simulink model "Full_network_time_optimized"  (R2025b)
settings: Solver=FixedStepAuto  StartTime=0.0  StopTime=30  FixedStep=0.001  RelTol=1e-3
InitFcn:
  | load('FuelPropsData.mat')
libraries: fl_lib x41, nesl_utility x31, SimscapeFluids_lib x13, slpidlib x7, simulink x4
(part 5 of 5)

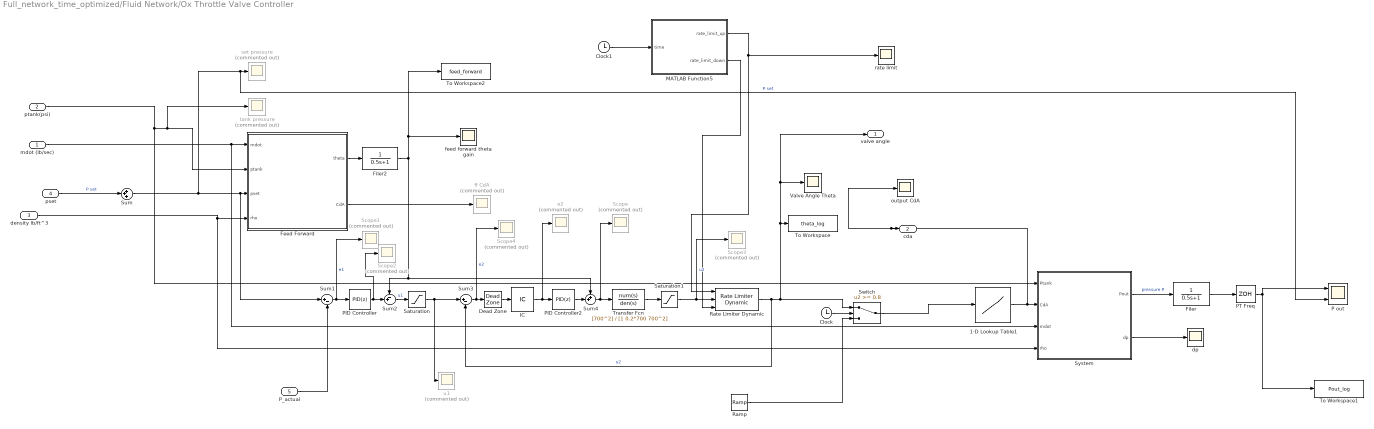
== system Full_network_time_optimized/Fluid Network/Ox Throttle Valve Controller ==
  mdot (lb/sec) : Inport
  ptank(psi) : Inport  Port=2
  density lb/ft^3 : Inport  Port=3
  pset : Inport  Port=4
  P_actual : Inport  Port=5
  1-D Lookup Table1 : Lookup_n-D  NumberOfTableDimensions=1  BreakpointsForDimension1=[27, 36, 45, 54, 63, 72, 81, 90]  Table="[0.01,  0.06, 0.21, 0.46, 0.83, 1.35, 2.04, 2.93] ./ 37.97"  ExtrapMethod=Clip  InternalRulePriority=Speed  RndMeth=Simplest
  Clock : Clock
  Clock1 : Clock
  Dead Zone : DeadZone  LowerValue=-30  UpperValue=30
  Feed Forward : MATLAB Function  TreatAsAtomicUnit=on
  Filer : TransferFcn  Denominator=[0.5 1]
  Filer2 : TransferFcn  Denominator=[0.5 1]
  IC : InitialCondition  Value=0
  MATLAB Function5 : MATLAB Function  TreatAsAtomicUnit=on
  P out : Scope  NumInputPorts=2
      settings: ActiveDisplayYMinimum=-31.526205571372174  ActiveDisplayYMaximum=283.73585014234965  DataLoggingVariableName=ScopeData20
  PID Controller : slpidlib/PID Controller  Controller=PID  Form=Parallel  TimeDomain=Discrete-time  UseExternalTs=off  SampleTime=0.01  IntegratorMethod=Forward Euler  FilterMethod=Forward Euler  ControllerParametersSource=internal  P=6  I=0.5  UseKiTs=off  D=0  UseExternalDerivativeSource=off  N=100  UseFilter=on  TunerSelectOption=Transfer Function Based (PID Tuner App)  InitialConditionSource=internal  InitialConditionForIntegrator=0  InitialConditionForFilter=0  DifferentiatorICPrevScaledInput=0  ExternalReset=none  TrackingMode=off  Kt=1  LimitOutput=off  SatLimitsSource=internal  UpperSaturationLimit=inf  LowerSaturationLimit=-inf  LinearizeAsGain=on  AntiWindupMode=none  Kb=1  LimitIntegrator=off  UpperIntegratorSaturationLimit=inf  LowerIntegratorSaturationLimit=-inf  POutMin=[]  POutMax=[]  IOutMin=[]  IOutMax=[]  DOutMin=[]  DOutMax=[]  NOutMin=[]  NOutMax=[]  SumOutMin=[]  SumOutMax=[]  SaturationOutMin=[]  SaturationOutMax=[]  PParamMin=[]  PParamMax=[]  IParamMin=[]  IParamMax=[]  DParamMin=[]  DParamMax=[]  NParamMin=[]  NParamMax=[]  KbParamMin=[]  KbParamMax=[]  KtParamMin=[]  KtParamMax=[]  KbOutMin=[]  KbOutMax=[]  KtOutMin=[]  KtOutMax=[]  IntegratorOutMin=[]  IntegratorOutMax=[]  FilterOutMin=[]  FilterOutMax=[]  SumI1OutMin=[]  SumI1OutMax=[]  SumI2OutMin=[]  SumI2OutMax=[]  SumI3OutMin=[]  SumI3OutMax=[]  SumI4OutMin=[]  SumI4OutMax=[]  SumDOutMin=[]  SumDOutMax=[]  DifferentiatorOutMin=[]  DifferentiatorOutMax=[]  FilterDiffOutCoefMin=[]  FilterDiffOutCoefMax=[]  ReciprocalOutMin=[]  ReciprocalOutMax=[]  SumDenOutMin=[]  SumDenOutMax=[]  SumNumOutMin=[]  SumNumOutMax=[]  DivideOutMin=[]  DivideOutMax=[]  UdiffTsProdOutMin=[]  UdiffTsProdOutMax=[]  NTsProdOutMin=[]  NTsProdOutMax=[]  UintegralTsProdOutMin=[]  UintegralTsProdOutMax=[]  UngainTsProdOutMin=[]  UngainTsProdOutMax=[]  ClampingZeroOutDataTypeStr=Inherit: Inherit via back propagation  ClampingZeroOutMin=[]  ClampingZeroOutMax=[]  FilterDenConstantOutDataTypeStr=Inherit: Inherit via back propagation  FilterDenConstantOutMin=[]  FilterDenConstantOutMax=[]  PCopyOutDataTypeStr=Inherit: Inherit via back propagation  PCopyOutMin=[]  PCopyOutMax=[]  NCopyOutDataTypeStr=Inherit: Inherit via back propagation  NCopyOutMin=[]  NCopyOutMax=[]  IntegratorContinuousStateAttributes=''  IntegratorStateMustResolveToSignalObject=off  IntegratorRTWStateStorageClass=Auto  FilterContinuousStateAttributes=''  FilterStateMustResolveToSignalObject=off  FilterRTWStateStorageClass=Auto  ParallelPVariant=InternalParameters  IdealPVariant=Disabled  IVariant=InternalParameters  DVariant=InternalParameters  IntegratorVariant=Discrete  SatVariant=Disabled  AWVariant=Passthrough  PCopyVariant=Disabled  TRVariant=Disabled  FdbkBlocksVariant=Forward  IdealPFdbkVariant=Disabled  SatFdbkVariant=Disabled  DerivativeFilterVariant=ForwardEulerFilter  NVariant=InternalParameters  NCopyVariant=Disabled  FilterICVariant=InternalICsFilter  IntegratorICVariant=InternalICs  ExternalResetVariant=Disabled  TRSumVariant=Passthrough  SumFdbkVariant=Disabled  SumVariant=Sum_PID  TsampFilterVariant=InternalTs  TsampNgainVariant=Passthrough  TsampIntegralVariant=Disabled_SignalSpec  ExternalSaturationOutDataTypeStr=Inherit: Same as second input  DerivativeSourceVariant=ErrorSignal  PreIntVariant=InternalPreInt
  PID Controller2 : slpidlib/PID Controller  Controller=PID  Form=Parallel  TimeDomain=Discrete-time  UseExternalTs=off  SampleTime=0.001  IntegratorMethod=Forward Euler  FilterMethod=Forward Euler  ControllerParametersSource=internal  P=0.1  I=0.6  UseKiTs=off  D=0  UseExternalDerivativeSource=off  N=100  UseFilter=on  TunerSelectOption=Transfer Function Based (PID Tuner App)  InitialConditionSource=internal  InitialConditionForIntegrator=0  InitialConditionForFilter=0  DifferentiatorICPrevScaledInput=0  ExternalReset=none  TrackingMode=off  Kt=1  LimitOutput=off  SatLimitsSource=internal  UpperSaturationLimit=inf  LowerSaturationLimit=-inf  LinearizeAsGain=on  AntiWindupMode=none  Kb=1  LimitIntegrator=off  UpperIntegratorSaturationLimit=inf  LowerIntegratorSaturationLimit=-inf  POutMin=[]  POutMax=[]  IOutMin=[]  IOutMax=[]  DOutMin=[]  DOutMax=[]  NOutMin=[]  NOutMax=[]  SumOutMin=[]  SumOutMax=[]  SaturationOutMin=[]  SaturationOutMax=[]  PParamMin=[]  PParamMax=[]  IParamMin=[]  IParamMax=[]  DParamMin=[]  DParamMax=[]  NParamMin=[]  NParamMax=[]  KbParamMin=[]  KbParamMax=[]  KtParamMin=[]  KtParamMax=[]  KbOutMin=[]  KbOutMax=[]  KtOutMin=[]  KtOutMax=[]  IntegratorOutMin=[]  IntegratorOutMax=[]  FilterOutMin=[]  FilterOutMax=[]  SumI1OutMin=[]  SumI1OutMax=[]  SumI2OutMin=[]  SumI2OutMax=[]  SumI3OutMin=[]  SumI3OutMax=[]  SumI4OutMin=[]  SumI4OutMax=[]  SumDOutMin=[]  SumDOutMax=[]  DifferentiatorOutMin=[]  DifferentiatorOutMax=[]  FilterDiffOutCoefMin=[]  FilterDiffOutCoefMax=[]  ReciprocalOutMin=[]  ReciprocalOutMax=[]  SumDenOutMin=[]  SumDenOutMax=[]  SumNumOutMin=[]  SumNumOutMax=[]  DivideOutMin=[]  DivideOutMax=[]  UdiffTsProdOutMin=[]  UdiffTsProdOutMax=[]  NTsProdOutMin=[]  NTsProdOutMax=[]  UintegralTsProdOutMin=[]  UintegralTsProdOutMax=[]  UngainTsProdOutMin=[]  UngainTsProdOutMax=[]  ClampingZeroOutDataTypeStr=Inherit: Inherit via back propagation  ClampingZeroOutMin=[]  ClampingZeroOutMax=[]  FilterDenConstantOutDataTypeStr=Inherit: Inherit via back propagation  FilterDenConstantOutMin=[]  FilterDenConstantOutMax=[]  PCopyOutDataTypeStr=Inherit: Inherit via back propagation  PCopyOutMin=[]  PCopyOutMax=[]  NCopyOutDataTypeStr=Inherit: Inherit via back propagation  NCopyOutMin=[]  NCopyOutMax=[]  IntegratorContinuousStateAttributes=''  IntegratorStateMustResolveToSignalObject=off  IntegratorRTWStateStorageClass=Auto  FilterContinuousStateAttributes=''  FilterStateMustResolveToSignalObject=off  FilterRTWStateStorageClass=Auto  ParallelPVariant=InternalParameters  IdealPVariant=Disabled  IVariant=InternalParameters  DVariant=InternalParameters  IntegratorVariant=Discrete  SatVariant=Disabled  AWVariant=Passthrough  PCopyVariant=Disabled  TRVariant=Disabled  FdbkBlocksVariant=Forward  IdealPFdbkVariant=Disabled  SatFdbkVariant=Disabled  DerivativeFilterVariant=ForwardEulerFilter  NVariant=InternalParameters  NCopyVariant=Disabled  FilterICVariant=InternalICsFilter  IntegratorICVariant=InternalICs  ExternalResetVariant=Disabled  TRSumVariant=Passthrough  SumFdbkVariant=Disabled  SumVariant=Sum_PID  TsampFilterVariant=InternalTs  TsampNgainVariant=Passthrough  TsampIntegralVariant=Disabled_SignalSpec  ExternalSaturationOutDataTypeStr=Inherit: Same as second input  DerivativeSourceVariant=ErrorSignal  PreIntVariant=InternalPreInt
  PT Freq : ZeroOrderHold  SampleTime=1/200
  Ramp : simulink/Sources/Ramp  slope=48  start=0  InitialOutput=0
  Rate Limiter Dynamic : simulink/Discontinuities/Rate Limiter Dynamic
  Saturation : Saturate  UpperLimit=90  LowerLimit=0
  Saturation1 : Saturate  UpperLimit=90  LowerLimit=0
  Scope{,1..4} (5 alike) : Scope  Commented=on
      Scope settings: ActiveDisplayYMinimum=-275.11641924282065  ActiveDisplayYMaximum=563.35245614782866  DataLoggingVariableName=ScopeData23
      Scope1 settings: ActiveDisplayYMinimum=-63.640747784829  ActiveDisplayYMaximum=395.9600830872032  DataLoggingVariableName=ScopeData24
      Scope2 settings: ActiveDisplayYMinimum=-1  ActiveDisplayYMaximum=1  DataLoggingVariableName=ScopeData25
      Scope3 settings: ActiveDisplayYMinimum=-1  ActiveDisplayYMaximum=1  DataLoggingVariableName=ScopeData26
      Scope4 settings: ActiveDisplayYMinimum=-1  ActiveDisplayYMaximum=1  DataLoggingVariableName=ScopeData27
  Sum : Sum  Inputs=+++
  Sum1 : Sum  Inputs=|+-
  Sum2 : Sum  Inputs=-+|
  Sum3 : Sum  Inputs=|+-
  Sum4 : Sum  Inputs=++|
  Switch : Switch  Threshold=0.8  SaturateOnIntegerOverflow=off  InputSameDT=off
  System : MATLAB Function  TreatAsAtomicUnit=on
  To Workspace : ToWorkspace  VariableName=theta_log  SampleTime=-1
  To Workspace1 : ToWorkspace  VariableName=Pout_log  SaveFormat=Structure With Time  SampleTime=-1
  To Workspace2 : ToWorkspace  VariableName=feed_forward  SampleTime=-1
  Transfer Fcn : TransferFcn  Numerator=[700^2]  Denominator=[1 0.2*700 700^2]
  Valve Angle Theta : Scope
      settings: ActiveDisplayYMinimum=-6.3882474794481388  ActiveDisplayYMaximum=57.494227315033264
  dp : Scope
      settings: ActiveDisplayYMinimum=-1  ActiveDisplayYMaximum=1  DataLoggingVariableName=ScopeData28
  e2 : Scope  Commented=on
      settings: ActiveDisplayYMinimum=-94.713391249832966  ActiveDisplayYMaximum=253.61308310962266  DataLoggingVariableName=ScopeData29
  feed forward theta gain : Scope
      settings: ActiveDisplayYMinimum=36.144112332478429  ActiveDisplayYMaximum=40.8018145520034  DataLoggingVariableName=ScopeData2
  ff CdA : Scope  Commented=on
      settings: ActiveDisplayYMinimum=0.00619  ActiveDisplayYMaximum=0.00757  DataLoggingVariableName=ScopeData30
  output CdA : Scope
      settings: ActiveDisplayYMinimum=-0.00091146165836572817  ActiveDisplayYMaximum=0.010836813076463534  DataLoggingVariableName=ScopeData3
  rate limit : Scope
      settings: ActiveDisplayYMinimum=-123.74999999999997  ActiveDisplayYMaximum=1513.75  DataLoggingVariableName=ScopeData31
  set pressure : Scope  Commented=on
      settings: ActiveDisplayYMinimum=-1  ActiveDisplayYMaximum=1  DataLoggingVariableName=ScopeData32
  tank pressure : Scope  Commented=on
      settings: ActiveDisplayYMinimum=243.75  ActiveDisplayYMaximum=306.25  DataLoggingVariableName=ScopeData33
  u1 : Scope  Commented=on
      settings: ActiveDisplayYMinimum=-1  ActiveDisplayYMaximum=1  DataLoggingVariableName=ScopeData34
  valve angle : Outport
  cda : Outport  Port=2
  wires:
  Sum3/1 -> Dead Zone/1, Scope4/1  "e2"
  density lb/ft^3/1 -> System/4(rho), Feed Forward/4(rho)
  Filer/1 -> PT Freq/1
  Sum/1 -> P out/2, set pressure/1, Sum1/1, Feed Forward/3(pset)  "P set"
  ptank(psi)/1 -> System/1(Ptank), Feed Forward/2(ptank), tank pressure/1
  PID Controller/1 -> Scope2/1, Sum2/2
  PT Freq/1 -> P out/1, To Workspace1/1
  Transfer Fcn/1 -> Saturation1/1
  IC/1 -> PID Controller2/1, e2/1
  Feed Forward/1(theta) -> Filer2/1
  MATLAB Function5/2(rate_limit_down) -> Rate Limiter Dynamic/3
  Dead Zone/1 -> IC/1
  Rate Limiter Dynamic/1 -> Switch/1, valve angle/1, Valve Angle Theta/1, To Workspace/1, Sum3/2  "u2"
  pset/1 -> Sum/2  "P set"
  Sum4/1 -> Scope/1, Transfer Fcn/1
  Saturation1/1 -> Scope3/1, Rate Limiter Dynamic/2  "u2"
  mdot (lb/sec)/1 -> System/3(mdot), Feed Forward/1(mdot)
  MATLAB Function5/1(rate_limit_up) -> Rate Limiter Dynamic/1, rate limit/1
  Clock1/1 -> MATLAB Function5/1(time)
  1-D Lookup Table1/1 -> System/2(CdA), output CdA/1, cda/1
  PID Controller2/1 -> Sum4/2
  Sum1/1 -> Scope1/1, PID Controller/1  "e1"
  Sum2/1 -> Saturation/1  "u1"
  Feed Forward/2(CdA) -> ff CdA/1
  System/2(dp) -> dp/1
  Saturation/1 -> u1/1, Sum3/1
  System/1(Pout) -> Filer/1  "pressure P"
  Filer2/1 -> Sum4/1, Sum2/1, feed forward theta gain/1, To Workspace2/1
  P_actual/1 -> Sum1/2
  Clock/1 -> Switch/2
  Ramp/1 -> Switch/3
  Switch/1 -> 1-D Lookup Table1/1

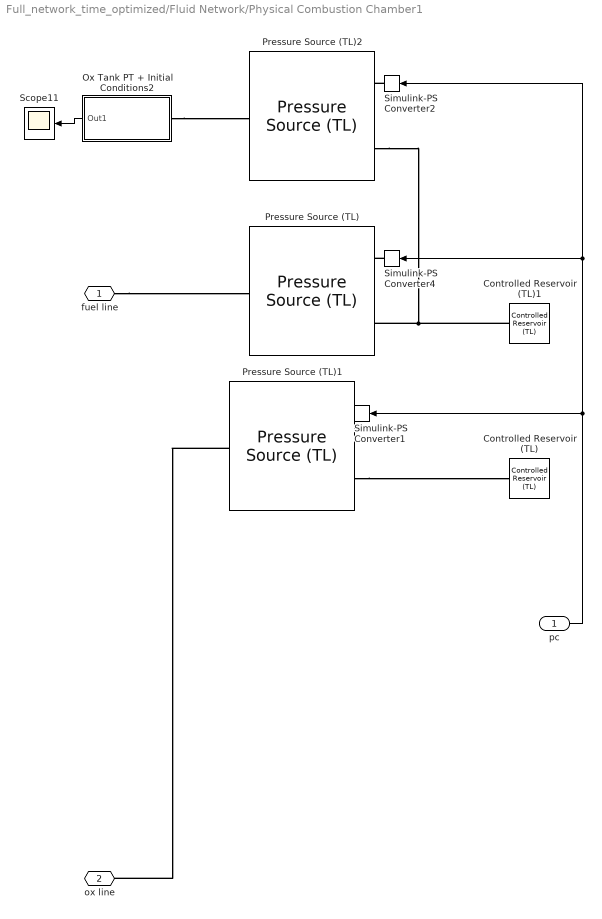
== system Full_network_time_optimized/Fluid Network/Physical Combustion Chamber1 ==
  pc : Inport
  Controlled Reservoir (TL) : fl_lib/Thermal Liquid/Elements/Controlled Reservoir (TL)  pressure_spec=foundation.enum.pressure_spec.atmospheric  reservoir_pressure=0.101325 MPa  area=0.01 m^2
      settings: InternalSimscapePortConfiguration="{\"Bottom\":[],\"Left\":[{\"id\":\"A\",\"label\":\"A\",\"type\":\"foundation.thermal_liquid.thermal_liquid\"}],\"Right\":[{\"id\":\"T_in\",\"label\":\"T\",\"type\":\"input\"}],\"Top\":[]}"
  Controlled Reservoir (TL)1 : fl_lib/Thermal Liquid/Elements/Controlled Reservoir (TL)  pressure_spec=foundation.enum.pressure_spec.atmospheric  reservoir_pressure=0.101325 MPa  area=0.01 m^2
      settings: InternalSimscapePortConfiguration="{\"Bottom\":[],\"Left\":[{\"id\":\"A\",\"label\":\"A\",\"type\":\"foundation.thermal_liquid.thermal_liquid\"}],\"Right\":[{\"id\":\"T_in\",\"label\":\"T\",\"type\":\"input\"}],\"Top\":[]}"
  Ox Tank PT + Initial Conditions2 : Subsystem
  Pressure Source (TL) : fl_lib/Thermal Liquid/Sources/Pressure Source (TL)  source_type=foundation.enum.constant_controlled.controlled  pressure_differential=0 MPa  power_spec=foundation.enum.power_spec.isentropic  area=0.01 m^2
      settings: InternalSimscapePortConfiguration="{\"Bottom\":[],\"Left\":[{\"id\":\"A\",\"label\":\"A\",\"type\":\"foundation.thermal_liquid.thermal_liquid\"},{\"id\":\"P\",\"label\":\"P\",\"type\":\"input\"}],\"Right\":[{\"id\":\"B\",\"label\":\"B\",\"type\":\"foundation.thermal_liquid.thermal_liquid\"}],\"Top\":[]}"
  Pressure Source (TL)1 : fl_lib/Thermal Liquid/Sources/Pressure Source (TL)  source_type=foundation.enum.constant_controlled.controlled  pressure_differential=0 MPa  power_spec=foundation.enum.power_spec.isentropic  area=0.01 m^2
      settings: InternalSimscapePortConfiguration="{\"Bottom\":[],\"Left\":[{\"id\":\"A\",\"label\":\"A\",\"type\":\"foundation.thermal_liquid.thermal_liquid\"},{\"id\":\"P\",\"label\":\"P\",\"type\":\"input\"}],\"Right\":[{\"id\":\"B\",\"label\":\"B\",\"type\":\"foundation.thermal_liquid.thermal_liquid\"}],\"Top\":[]}"
  Pressure Source (TL)2 : fl_lib/Thermal Liquid/Sources/Pressure Source (TL)  source_type=foundation.enum.constant_controlled.controlled  pressure_differential=0 MPa  power_spec=foundation.enum.power_spec.isentropic  area=0.01 m^2
      settings: InternalSimscapePortConfiguration="{\"Bottom\":[],\"Left\":[{\"id\":\"A\",\"label\":\"A\",\"type\":\"foundation.thermal_liquid.thermal_liquid\"},{\"id\":\"P\",\"label\":\"P\",\"type\":\"input\"}],\"Right\":[{\"id\":\"B\",\"label\":\"B\",\"type\":\"foundation.thermal_liquid.thermal_liquid\"}],\"Top\":[]}"
  Scope11 : Scope
      settings: ActiveDisplayYMinimum=-62.499971643181354  ActiveDisplayYMaximum=562.49999684924239  DataLoggingVariableName=ScopeData48
  Simulink-PS Converter1 : nesl_utility/Simulink-PS Converter  PhysicalDomain=network_engine_domain  SubClassName=ps_input  LeftPortType=input  RightPortType=output  PseudoPeriodic=off  Frequencies=[]  NoiseDistribution=none  NoiseParameters=[]  Unit=1  AffineConversion=off  FilteringAndDerivatives=filter  SimscapeFilterOrder=1  InputFilterTimeConstant=0.001  UdotUserProvided=0
  Simulink-PS Converter2 : nesl_utility/Simulink-PS Converter  PhysicalDomain=network_engine_domain  SubClassName=ps_input  LeftPortType=input  RightPortType=output  PseudoPeriodic=off  Frequencies=[]  NoiseDistribution=none  NoiseParameters=[]  Unit=1  AffineConversion=off  FilteringAndDerivatives=filter  SimscapeFilterOrder=1  InputFilterTimeConstant=0.001  UdotUserProvided=0
  Simulink-PS Converter4 : nesl_utility/Simulink-PS Converter  PhysicalDomain=network_engine_domain  SubClassName=ps_input  LeftPortType=input  RightPortType=output  PseudoPeriodic=off  Frequencies=[]  NoiseDistribution=none  NoiseParameters=[]  Unit=1  AffineConversion=off  FilteringAndDerivatives=filter  SimscapeFilterOrder=1  InputFilterTimeConstant=0.001  UdotUserProvided=0
  fuel line : PMIOPort  Side=Right
  ox line : PMIOPort  Port=2  Side=Right
  wires:
  pc/1 -> Simulink-PS Converter1/1, Simulink-PS Converter2/1, Simulink-PS Converter4/1
  Ox Tank PT + Initial Conditions2/1(Out1) -> Scope11/1
  connections:
  Simulink-PS Converter4/RConn1 -- Pressure Source (TL)/LConn2
  Simulink-PS Converter1/RConn1 -- Pressure Source (TL)1/LConn2
  Controlled Reservoir (TL)1/LConn1 -- Pressure Source (TL)2/LConn1 -- Pressure Source (TL)/LConn1
  fuel line/RConn1 -- Pressure Source (TL)/RConn1
  Pressure Source (TL)1/RConn1 -- ox line/RConn1
  Pressure Source (TL)1/LConn1 -- Controlled Reservoir (TL)/LConn1
  Simulink-PS Converter2/RConn1 -- Pressure Source (TL)2/LConn2
  Ox Tank PT + Initial Conditions2/LConn1 -- Pressure Source (TL)2/RConn1

== system Full_network_time_optimized/Fluid Network/fuel mdot feedback//corrections ==
  actual mdot : Inport
  commanded mdot : Inport  Port=2
  MR correction : Inport  Port=3
  PID Controller1 : slpidlib/PID Controller  Controller=PID  Form=Parallel  TimeDomain=Continuous-time  UseExternalTs=off  SampleTime=-1  IntegratorMethod=Forward Euler  FilterMethod=Forward Euler  ControllerParametersSource=internal  P=1  I=0  UseKiTs=off  D=0  UseExternalDerivativeSource=off  N=20  UseFilter=on  TunerSelectOption=Transfer Function Based (PID Tuner App)  InitialConditionSource=internal  InitialConditionForIntegrator=0  InitialConditionForFilter=0  DifferentiatorICPrevScaledInput=0  ExternalReset=none  TrackingMode=off  Kt=1  LimitOutput=off  SatLimitsSource=internal  UpperSaturationLimit=inf  LowerSaturationLimit=-inf  LinearizeAsGain=on  AntiWindupMode=none  Kb=1  LimitIntegrator=off  UpperIntegratorSaturationLimit=inf  LowerIntegratorSaturationLimit=-inf  POutMin=[]  POutMax=[]  IOutMin=[]  IOutMax=[]  DOutMin=[]  DOutMax=[]  NOutMin=[]  NOutMax=[]  SumOutMin=[]  SumOutMax=[]  SaturationOutMin=[]  SaturationOutMax=[]  PParamMin=[]  PParamMax=[]  IParamMin=[]  IParamMax=[]  DParamMin=[]  DParamMax=[]  NParamMin=[]  NParamMax=[]  KbParamMin=[]  KbParamMax=[]  KtParamMin=[]  KtParamMax=[]  KbOutMin=[]  KbOutMax=[]  KtOutMin=[]  KtOutMax=[]  IntegratorOutMin=[]  IntegratorOutMax=[]  FilterOutMin=[]  FilterOutMax=[]  SumI1OutMin=[]  SumI1OutMax=[]  SumI2OutMin=[]  SumI2OutMax=[]  SumI3OutMin=[]  SumI3OutMax=[]  SumI4OutMin=[]  SumI4OutMax=[]  SumDOutMin=[]  SumDOutMax=[]  DifferentiatorOutMin=[]  DifferentiatorOutMax=[]  FilterDiffOutCoefMin=[]  FilterDiffOutCoefMax=[]  ReciprocalOutMin=[]  ReciprocalOutMax=[]  SumDenOutMin=[]  SumDenOutMax=[]  SumNumOutMin=[]  SumNumOutMax=[]  DivideOutMin=[]  DivideOutMax=[]  UdiffTsProdOutMin=[]  UdiffTsProdOutMax=[]  NTsProdOutMin=[]  NTsProdOutMax=[]  UintegralTsProdOutMin=[]  UintegralTsProdOutMax=[]  UngainTsProdOutMin=[]  UngainTsProdOutMax=[]  ClampingZeroOutDataTypeStr=Inherit: Inherit via back propagation  ClampingZeroOutMin=[]  ClampingZeroOutMax=[]  FilterDenConstantOutDataTypeStr=Inherit: Inherit via back propagation  FilterDenConstantOutMin=[]  FilterDenConstantOutMax=[]  PCopyOutDataTypeStr=Inherit: Inherit via back propagation  PCopyOutMin=[]  PCopyOutMax=[]  NCopyOutDataTypeStr=Inherit: Inherit via back propagation  NCopyOutMin=[]  NCopyOutMax=[]  IntegratorContinuousStateAttributes=''  IntegratorStateMustResolveToSignalObject=off  IntegratorRTWStateStorageClass=Auto  FilterContinuousStateAttributes=''  FilterStateMustResolveToSignalObject=off  FilterRTWStateStorageClass=Auto  ParallelPVariant=InternalParameters  IdealPVariant=Disabled  IVariant=InternalParameters  DVariant=InternalParameters  IntegratorVariant=Continuous  SatVariant=Disabled  AWVariant=Passthrough  PCopyVariant=Disabled  TRVariant=Disabled  FdbkBlocksVariant=Forward  IdealPFdbkVariant=Disabled  SatFdbkVariant=Disabled  DerivativeFilterVariant=ContFilter  NVariant=InternalParameters  NCopyVariant=Disabled  FilterICVariant=InternalICsFilter  IntegratorICVariant=InternalICs  ExternalResetVariant=Disabled  TRSumVariant=Passthrough  SumFdbkVariant=Disabled  SumVariant=Sum_PID  TsampFilterVariant=InternalTs  TsampNgainVariant=Passthrough  TsampIntegralVariant=Disabled_SignalSpec  ExternalSaturationOutDataTypeStr=Inherit: Same as second input  DerivativeSourceVariant=ErrorSignal  PreIntVariant=InternalPreInt
  Sum2 : Sum  Inputs=|+-
  Sum3 : Sum  Inputs=|+-
  Sum4 : Sum  Inputs=|++
  kg/s to lb/s1 : Gain  Gain=2.20462
  fuel mdot : Outport
  wires:
  PID Controller1/1 -> Sum4/1
  Sum3/1 -> PID Controller1/1
  Sum4/1 -> kg/s to lb/s1/1
  commanded mdot/1 -> Sum2/1
  Sum2/1 -> Sum3/1
  MR correction/1 -> Sum3/2
  kg/s to lb/s1/1 -> fuel mdot/1

== system Full_network_time_optimized/Fluid Network/ox mdot feedback//corrections ==
  commanded mdot : Inport
  actual mdot : Inport  Port=2
  PID Controller2 : slpidlib/PID Controller  Commented=through  Controller=PID  Form=Parallel  TimeDomain=Continuous-time  UseExternalTs=off  SampleTime=-1  IntegratorMethod=Forward Euler  FilterMethod=Forward Euler  ControllerParametersSource=internal  P=1  I=0  UseKiTs=off  D=0  UseExternalDerivativeSource=off  N=20  UseFilter=on  TunerSelectOption=Transfer Function Based (PID Tuner App)  InitialConditionSource=internal  InitialConditionForIntegrator=0  InitialConditionForFilter=0  DifferentiatorICPrevScaledInput=0  ExternalReset=none  TrackingMode=off  Kt=1  LimitOutput=off  SatLimitsSource=internal  UpperSaturationLimit=inf  LowerSaturationLimit=-inf  LinearizeAsGain=on  AntiWindupMode=none  Kb=1  LimitIntegrator=off  UpperIntegratorSaturationLimit=inf  LowerIntegratorSaturationLimit=-inf  POutMin=[]  POutMax=[]  IOutMin=[]  IOutMax=[]  DOutMin=[]  DOutMax=[]  NOutMin=[]  NOutMax=[]  SumOutMin=[]  SumOutMax=[]  SaturationOutMin=[]  SaturationOutMax=[]  PParamMin=[]  PParamMax=[]  IParamMin=[]  IParamMax=[]  DParamMin=[]  DParamMax=[]  NParamMin=[]  NParamMax=[]  KbParamMin=[]  KbParamMax=[]  KtParamMin=[]  KtParamMax=[]  KbOutMin=[]  KbOutMax=[]  KtOutMin=[]  KtOutMax=[]  IntegratorOutMin=[]  IntegratorOutMax=[]  FilterOutMin=[]  FilterOutMax=[]  SumI1OutMin=[]  SumI1OutMax=[]  SumI2OutMin=[]  SumI2OutMax=[]  SumI3OutMin=[]  SumI3OutMax=[]  SumI4OutMin=[]  SumI4OutMax=[]  SumDOutMin=[]  SumDOutMax=[]  DifferentiatorOutMin=[]  DifferentiatorOutMax=[]  FilterDiffOutCoefMin=[]  FilterDiffOutCoefMax=[]  ReciprocalOutMin=[]  ReciprocalOutMax=[]  SumDenOutMin=[]  SumDenOutMax=[]  SumNumOutMin=[]  SumNumOutMax=[]  DivideOutMin=[]  DivideOutMax=[]  UdiffTsProdOutMin=[]  UdiffTsProdOutMax=[]  NTsProdOutMin=[]  NTsProdOutMax=[]  UintegralTsProdOutMin=[]  UintegralTsProdOutMax=[]  UngainTsProdOutMin=[]  UngainTsProdOutMax=[]  ClampingZeroOutDataTypeStr=Inherit: Inherit via back propagation  ClampingZeroOutMin=[]  ClampingZeroOutMax=[]  FilterDenConstantOutDataTypeStr=Inherit: Inherit via back propagation  FilterDenConstantOutMin=[]  FilterDenConstantOutMax=[]  PCopyOutDataTypeStr=Inherit: Inherit via back propagation  PCopyOutMin=[]  PCopyOutMax=[]  NCopyOutDataTypeStr=Inherit: Inherit via back propagation  NCopyOutMin=[]  NCopyOutMax=[]  IntegratorContinuousStateAttributes=''  IntegratorStateMustResolveToSignalObject=off  IntegratorRTWStateStorageClass=Auto  FilterContinuousStateAttributes=''  FilterStateMustResolveToSignalObject=off  FilterRTWStateStorageClass=Auto  ParallelPVariant=InternalParameters  IdealPVariant=Disabled  IVariant=InternalParameters  DVariant=InternalParameters  IntegratorVariant=Continuous  SatVariant=Disabled  AWVariant=Passthrough  PCopyVariant=Disabled  TRVariant=Disabled  FdbkBlocksVariant=Forward  IdealPFdbkVariant=Disabled  SatFdbkVariant=Disabled  DerivativeFilterVariant=ContFilter  NVariant=InternalParameters  NCopyVariant=Disabled  FilterICVariant=InternalICsFilter  IntegratorICVariant=InternalICs  ExternalResetVariant=Disabled  TRSumVariant=Passthrough  SumFdbkVariant=Disabled  SumVariant=Sum_PID  TsampFilterVariant=InternalTs  TsampNgainVariant=Passthrough  TsampIntegralVariant=Disabled_SignalSpec  ExternalSaturationOutDataTypeStr=Inherit: Same as second input  DerivativeSourceVariant=ErrorSignal  PreIntVariant=InternalPreInt
  Sum1 : Sum  Inputs=|+-
  Sum5 : Sum  Inputs=|++
  kg/s to lb/s : Gain  Gain=2.20462
  ox mdot : Outport
  wires:
  Sum1/1 -> PID Controller2/1
  commanded mdot/1 -> Sum1/1
  PID Controller2/1 -> Sum5/1
  Sum5/1 -> kg/s to lb/s/1
  kg/s to lb/s/1 -> ox mdot/1

== system Full_network_time_optimized/Fluid Network/COPV/COPV Leakage ==
  Leak Rate : fl_lib/Gas/Elements/Flow Resistance (G)  delta_p_nominal=0.001 MPa  mdot_nominal=0.0000000001 kg/s  rho_nominal=0 kg/m^3  area=0.01 m^2  laminar_fraction=1e-3
      settings: InternalSimscapePortConfiguration="{\"Bottom\":[],\"Left\":[{\"id\":\"A\",\"label\":\"A\",\"type\":\"foundation.gas.gas\"}],\"Right\":[{\"id\":\"B\",\"label\":\"B\",\"type\":\"foundation.gas.gas\"}],\"Top\":[]}"
  Mass & Energy Flow Rate Sensor (G)2 : fl_lib/Gas/Sensors/Flow Rate Sensor (G)  mass_flow_measure=true  volumetric_flow_measure=false  volumetric_flow_conditions=foundation.enum.volumetric_flow_conditions.actual  p_std=0.101325 MPa  T_std=20 degC  energy_flow_measure=true
      settings: InternalSimscapePortConfiguration="{\"Bottom\":[{\"id\":\"PHI\",\"label\":\"φ\",\"type\":\"output\"}],\"Left\":[{\"id\":\"A\",\"label\":\"A\",\"type\":\"foundation.gas.gas\"}],\"Right\":[{\"id\":\"B\",\"label\":\"B\",\"type\":\"foundation.gas.gas\"},{\"id\":\"M\",\"label\":\"M\",\"type\":\"output\"}],\"Top\":[]}"
  PS-Simulink Converter7 : nesl_utility/PS-Simulink Converter  PhysicalDomain=network_engine_domain  SubClassName=ps_output  LeftPortType=input  RightPortType=output  PseudoPeriodic=off  Frequencies=[]  VectorFormat=inherit  Unit=inherit  AffineConversion=off
  Pressurant Mass Leak Rate : Scope  Commented=on
      settings: ActiveDisplayYMinimum=-1  ActiveDisplayYMaximum=1
  Reservoir (G) : fl_lib/Gas/Elements/Reservoir (G)  pressure_spec=foundation.enum.pressure_spec.atmospheric  reservoir_pressure=0.101325 MPa  reservoir_temperature=293.15 K  area_A=0.01 m^2
  Conn1 : PMIOPort  Side=Right
  wires:
  PS-Simulink Converter7/1 -> Pressurant Mass Leak Rate/1
  connections:
  Conn1/RConn1 -- Leak Rate/RConn1
  Leak Rate/LConn1 -- Mass & Energy Flow Rate Sensor (G)2/LConn1
  Mass & Energy Flow Rate Sensor (G)2/RConn1 -- Reservoir (G)/LConn1
  Mass & Energy Flow Rate Sensor (G)2/RConn2 -- PS-Simulink Converter7/LConn1

== system Full_network_time_optimized/Fluid Network/Physical Combustion Chamber1/Ox Tank PT + Initial Conditions2 ==
  Initial OT Pressure : InitialCondition  Value=500
  PS-Simulink Converter3 : nesl_utility/PS-Simulink Converter  PhysicalDomain=network_engine_domain  SubClassName=ps_output  LeftPortType=input  RightPortType=output  PseudoPeriodic=off  Frequencies=[]  VectorFormat=inherit  Unit=inherit  AffineConversion=off
  Pa to psi : Gain  Gain=0.000145038
  Pressure & Temperature Sensor (TL) : fl_lib/Thermal Liquid/Sensors/Pressure & Temperature Sensor (TL)  reference=foundation.enum.MeasurementReference.absolute  pressure=true  pressure_spec=foundation.enum.PressureMeasementSpec.Gauge  temperature=false
      settings: InternalSimscapePortConfiguration="{\"Bottom\":[],\"Left\":[{\"id\":\"A\",\"label\":\"A\",\"type\":\"foundation.thermal_liquid.thermal_liquid\"}],\"Right\":[{\"id\":\"Pg\",\"label\":\"Pg\",\"type\":\"output\"}],\"Top\":[]}"
  fuel line : PMIOPort  Side=Left
  Out1 : Outport
  wires:
  Initial OT Pressure/1 -> Out1/1
  Pa to psi/1 -> Initial OT Pressure/1
  PS-Simulink Converter3/1 -> Pa to psi/1
  connections:
  PS-Simulink Converter3/LConn1 -- Pressure & Temperature Sensor (TL)/RConn1
  Pressure & Temperature Sensor (TL)/LConn1 -- fuel line/RConn1

== matlab function Full_network_time_optimized/Fluid Network/Fuel Throttle Valve Controller/MATLAB Function5 ==
  data: time input; rate_limit_up output; rate_limit_down output
function [rate_limit_up, rate_limit_down] = fcn(time)
if time < 0.5
    rate_limit_up = 1350;
else
    rate_limit_up = 40;
end
rate_limit_down = -rate_limit_up;

== matlab function Full_network_time_optimized/Fluid Network/Fuel Throttle Valve Controller/System ==
  data: Ptank input; CdA input; mdot input; Pout output; rho input; dp output
function [Pout,dp] = theta_to_pressure(Ptank,CdA,mdot, rho)

% CdA = mdot/(sqrt((2*(ptank-pout)*rho)

%CdA = max(CdA, 1e-7);
dp = (mdot/CdA)^2*1/(2*rho);

% (mdot/CdA)^2*rho/2 is solving for the pout from the dp in CdA eqn
Pout = Ptank - dp;
Pout = max(Pout, 0);

== matlab function Full_network_time_optimized/Fluid Network/Injector1/Fuel Injector Calculations ==
  data: P_down input; rho input; mdot input; CdA input; stiffness output; P_up output; dP_inj output
function [stiffness, P_up, dP_inj] = injectorModel(P_down, rho, mdot, CdA)
%#codegen
% Injector model using known downstream pressure, density, mdot, and CdA
%
% Inputs:
%   P_down - Downstream / chamber pressure [Pa]
%   rho    - Fluid density [kg/m^3]
%   mdot   - Mass flow rate through injector [kg/s]
%   CdA    - Effective injector area, Cd*A [m^2]
%
% Outputs:
%   stiffness - Injector stiffness, S = dP_inj / P_down [-]
%   P_up      - Required upstream / manifold pressure [Pa]
%   dP_inj    - Pressure drop across injector [Pa]
%
% Equations:
%   mdot   = CdA * sqrt(2 * rho * dP_inj)
%   => dP_inj = (mdot / CdA)^2 / (2*rho)
%
%   P_up = P_down + dP_inj
%   stiffness = dP_inj / P_down

    % Compute pressure drop from orifice equation
    dP_inj = (mdot / CdA)^2 / (2 * rho);

    % Upstream pressure
    P_up = P_down + dP_inj;

    % Stiffness
    stiffness = dP_inj / P_down;

end

== matlab function Full_network_time_optimized/Fluid Network/Thrust Commanded to mdot + bunch of other bs ==
  data: mdot_fuel output; rho_fuel_eng output; pc output; F_cmd input; rho_ox input; rho_fuel input; rho_ox_eng output; mdot_ox output; Cf input; MR input; cstar_ideal input; cstar_eff input
function [mdot_fuel, rho_fuel_eng, pc, rho_ox_eng, mdot_ox] = thrust_to_mdot( ...
   F_cmd, rho_ox, rho_fuel, Cf, MR, cstar_ideal, cstar_eff)
%#codegen
% Convert commanded thrust into mdots and convert densities to English units
%
% Outputs:
%   mdot_ox        - oxidizer mass flow rate [kg/s]
%   mdot_fuel      - fuel mass flow rate [kg/s]
%   rho_ox_eng     - oxidizer density [lb/ft^3]
%   rho_fuel_eng   - fuel density [lb/ft^3]
%   mdot_ox_lb     - oxidizer mass flow rate [lb/s]
%   mdot_fuel_lb   - fuel mass flow rate [lb/s]

    cstar = cstar_ideal * cstar_eff;
    At = 0.0008271;      % throat area [m^2]

    %% ---- DEFAULT OUTPUTS ----
    mdot_ox = 0;
    mdot_fuel = 0;
    rho_ox_eng = 0;
    rho_fuel_eng = 0;
    mdot_ox_lb = 0;
    mdot_fuel_lb = 0;

    %% ---- UNIT CONVERSION ----
    kgm3_to_lbft3 = 0.062428;
    kg_to_lb = 2.20462;

    rho_ox_eng = rho_ox * kgm3_to_lbft3;
    rho_fuel_eng = rho_fuel * kgm3_to_lbft3;

    %% ---- EFFECTIVE EXHAUST VELOCITY ----
    ve = Cf * cstar;


    %% ---- TOTAL MASS FLOW ----
    mdot_total = F_cmd / ve;

    pc = mdot_total * cstar / At;

    pc = pc * 0.000145038;

    %% ---- SPLIT BY MR ----
    mdot_ox = mdot_total * MR / (1 + MR);
    mdot_fuel = mdot_total / (1 + MR);


end

== matlab function Full_network_time_optimized/Fluid Network/MATLAB Function ==
  data: mdot_ox input; mdot_fuel input; eta_cstar input; Cf input; thrust output; Pc output; MR output; cstar_ideal input; mdot output
function [thrust, Pc, MR, mdot] = engine_model(mdot_ox, mdot_fuel, eta_cstar, Cf, cstar_ideal)
%#codegen
% ENGINE_MODEL
%
% Inputs:
%   mdot_ox      - oxidizer mass flow rate [kg/s]
%   mdot_fuel    - fuel mass flow rate [kg/s]
%   eta_cstar    - c* efficiency [-]
%   Cf           - thrust coefficient [-]
%
% Outputs:
%   thrust       - thrust [N]
%   Pc           - chamber pressure [Pa]
%   MR           - mixture ratio [-]

    %% -------------------------
    % CONSTANTS
    % -------------------------
    At = 0.0008271;      % throat area [m^2]

    %% -------------------------
    % 1. Total mass flow
    % -------------------------
    mdot = mdot_ox + mdot_fuel;

    %% -------------------------
    % 2. Mixture ratio
    % -------------------------
    if mdot_fuel > 0
        MR = mdot_ox / mdot_fuel;
    else
        MR = 0; % avoid divide by zero
    end

    %% -------------------------
    % 3. Actual c*
    % -------------------------
    cstar_actual = eta_cstar * cstar_ideal;

    %% -------------------------
    % 4. Chamber pressure
    % -------------------------
    Pc = (mdot * cstar_actual) / At;

    %% -------------------------
    % 6. Thrust
    % -------------------------
    thrust = Cf * Pc * At;

    % Equivalent:
    % thrust = Cf * mdot * cstar_actual;

end

== matlab function Full_network_time_optimized/Fluid Network/Injector2/Ox Injector Calculations ==
  data: P_down input; rho input; mdot input; CdA input; stiffness output; P_up output; dP_inj output
function [stiffness, P_up, dP_inj] = injectorModel(P_down, rho, mdot, CdA)
%#codegen
% Injector model using known downstream pressure, density, mdot, and CdA
%
% Inputs:
%   P_down - Downstream / chamber pressure [Pa]
%   rho    - Fluid density [kg/m^3]
%   mdot   - Mass flow rate through injector [kg/s]
%   CdA    - Effective injector area, Cd*A [m^2]
%
% Outputs:
%   stiffness - Injector stiffness, S = dP_inj / P_down [-]
%   P_up      - Required upstream / manifold pressure [Pa]
%   dP_inj    - Pressure drop across injector [Pa]
%
% Equations:
%   mdot   = CdA * sqrt(2 * rho * dP_inj)
%   => dP_inj = (mdot / CdA)^2 / (2*rho)
%
%   P_up = P_down + dP_inj
%   stiffness = dP_inj / P_down

    % Compute pressure drop from orifice equation
    dP_inj = (mdot / CdA)^2 / (2 * rho);

    % Upstream pressure
    P_up = P_down + dP_inj;

    % Stiffness
    stiffness = dP_inj / P_down;

end

== matlab function Full_network_time_optimized/Fluid Network/Fuel Throttle Valve Controller/Feed Forward ==
  data: mdot input; theta output; ptank input; pset input; rho input; CdA output
function [theta, CdA] = feed_forward(mdot,ptank,pset,rho)

dp = max(ptank - pset, 1e-6); % divide by zero erro

rho = max(rho, 1e-6);
CdA = mdot / sqrt(2*dp*rho);

CdA = max(CdA, 1e-7); % divide by zero error
Cv_vector = [1e-8, 0.01, 0.06, 0.21, 0.46, 0.83, 1.35, 2.04, 2.93];
CdA_vector = Cv_vector ./ 37.97;
theta_vector = 0.9.*[20,30,40,50,60,70,80,90,100];

theta = interp1(CdA_vector, theta_vector, CdA);
theta = min(theta, 90);
theta = max(theta, 0);
end

== matlab function Full_network_time_optimized/Fluid Network/Ox Throttle Valve Controller/Feed Forward ==
  data: mdot input; theta output; ptank input; pset input; rho input; CdA output
function [theta, CdA] = feed_forward(mdot,ptank,pset,rho)

dp = max(ptank - pset, 1e-6); % divide by zero erro

rho = max(rho, 1e-6);
CdA = mdot / sqrt(2*dp*rho);

CdA = max(CdA, 1e-7); % divide by zero error
Cv_vector = [1e-8, 0.01, 0.06, 0.21, 0.46, 0.83, 1.35, 2.04, 2.93];
CdA_vector = Cv_vector ./ 37.97;
theta_vector = 0.9.*[20,30,40,50,60,70,80,90,100];

theta = interp1(CdA_vector, theta_vector, CdA);
theta = min(theta, 90);
theta = max(theta, 0);
end

== matlab function Full_network_time_optimized/Fluid Network/Ox Throttle Valve Controller/MATLAB Function5 ==
  data: time input; rate_limit_up output; rate_limit_down output
function [rate_limit_up, rate_limit_down] = fcn(time)
if time < 0.5
    rate_limit_up = 1350;
else
    rate_limit_up = 40;
end
rate_limit_down = -rate_limit_up;

== matlab function Full_network_time_optimized/Fluid Network/Ox Throttle Valve Controller/System ==
  data: Ptank input; CdA input; mdot input; Pout output; rho input; dp output
function [Pout,dp] = theta_to_pressure(Ptank,CdA,mdot, rho)

% CdA = mdot/(sqrt((2*(ptank-pout)*rho)

%CdA = max(CdA, 1e-7);
dp = (mdot/CdA)^2*1/(2*rho);

% (mdot/CdA)^2*rho/2 is solving for the pout from the dp in CdA eqn
Pout = Ptank - dp;
Pout = max(Pout, 0);
